simulink model "BigBen_Controller_Test"  (R2025b)
settings: Solver=ode45
settings Model: Creator=Compu  LastModifiedBy=ahmed medhat

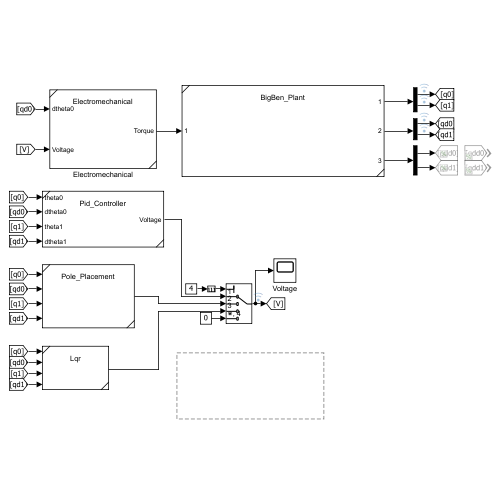
[thumbnail: Simulink's stored preview of the top-level diagram]
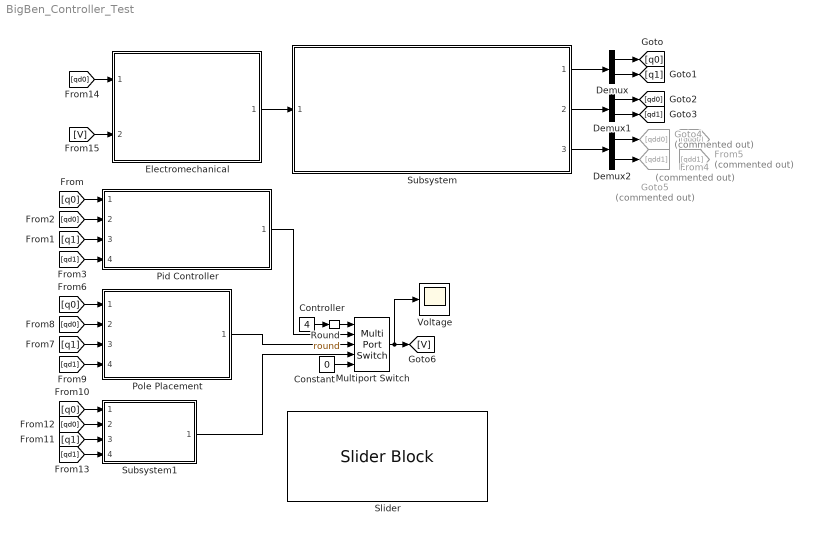
== system BigBen_Controller_Test ==
  Constant : Constant  Value=0
  Controller : Constant  Value=4
  Demux : Demux  Outputs=2
  Demux1 : Demux  Outputs=2
  Demux2 : Demux  Outputs=2
  Electromechanical : Subsystem  ReferencedSubsystem=Electromechanical
  From4 : From  Commented=on  GotoTag=qdd0
  From5 : From  Commented=on  GotoTag=qdd1
  Goto4 : Goto  Commented=on  GotoTag=qdd0
  Goto5 : Goto  Commented=on  GotoTag=qdd1
  Multiport Switch : MultiPortSwitch  Inputs=4  SaturateOnIntegerOverflow=off  InputSameDT=off
  Pid Controller : Subsystem  ReferencedSubsystem=Pid_Controller
  Pole Placement : Subsystem  ReferencedSubsystem=Pole_Placement
  Round : Rounding  Operator=round
  Slider : SliderBlock  ScaleMin=1  ScaleMax=4  TickInterval=1
  Subsystem : Subsystem  ReferencedSubsystem=BigBen_Plant
  Subsystem1 : Subsystem  ReferencedSubsystem=Lqr
  Voltage : Scope
      settings: ActiveDisplayYMinimum=-3.2199569205274443  ActiveDisplayYMaximum=0.60844546471572569  DataLoggingVariableName=ScopeData4
  wires:
  Subsystem/1 -> Demux/1
  Subsystem/2 -> Demux1/1
  Subsystem/3 -> Demux2/1
  Demux/1 -> [q0]
  Demux/2 -> [q1]
  Demux1/1 -> [qd0]
  Demux1/2 -> [qd1]
  Demux2/1 -> Goto4/1
  Demux2/2 -> Goto5/1
  [q0] -> Pid Controller/1
  [q1] -> Pid Controller/3
  [qd0] -> Pid Controller/2
  [qd1] -> Pid Controller/4
  [q0] -> Pole Placement/1
  [qd0] -> Pole Placement/2
  [q1] -> Pole Placement/3
  [qd1] -> Pole Placement/4
  Electromechanical/1 -> Subsystem/1
  [q1] -> Subsystem1/3
  [qd0] -> Subsystem1/2
  [q0] -> Subsystem1/1
  [qd1] -> Subsystem1/4
  [qd0] -> Electromechanical/1
  Pid Controller/1 -> Multiport Switch/2
  Pole Placement/1 -> Multiport Switch/3
  Subsystem1/1 -> Multiport Switch/4
  Multiport Switch/1 -> Voltage/1, [V]
  [V] -> Electromechanical/2
  Constant/1 -> Multiport Switch/5
  Round/1 -> Multiport Switch/1
  Controller/1 -> Round/1
